simulink model "parcial_2_simulaciones"  (R2026a)
settings: Solver=VariableStepAuto
undefined symbols (not defined in the file): A, B, C, D
settings Model: Creator=santi  LastModifiedBy=elkin

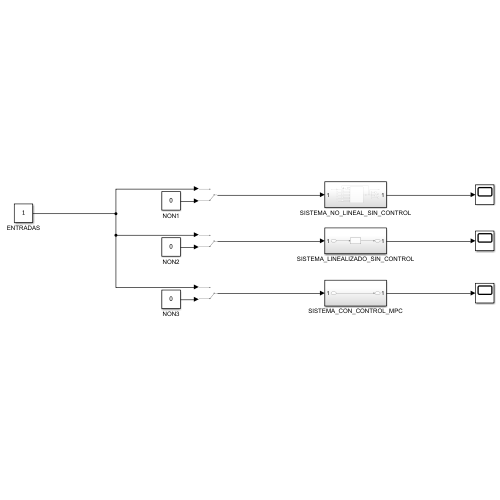
[thumbnail: Simulink's stored preview of the top-level diagram]
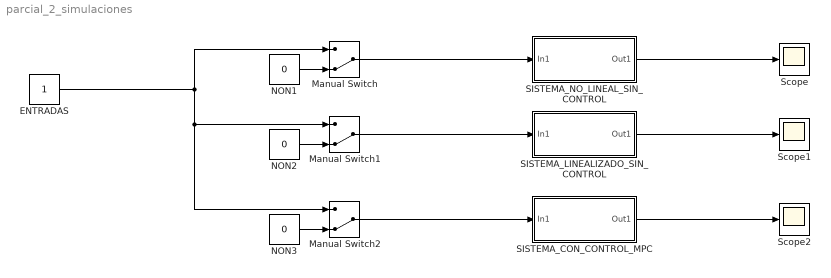
== system parcial_2_simulaciones ==
  ENTRADAS : Constant
  Manual Switch : ManualSwitch  CurrentSetting=0
  Manual Switch1 : ManualSwitch  CurrentSetting=0
  Manual Switch2 : ManualSwitch  CurrentSetting=0
  NON1 : Constant  Value=0
  NON2 : Constant  Value=0
  NON3 : Constant  Value=0
  SISTEMA_CON_CONTROL_MPC : Subsystem
  SISTEMA_LINEALIZADO_SIN_CONTROL : Subsystem
  SISTEMA_NO_LINEAL_SIN_CONTROL : Subsystem
  Scope : Scope
  Scope1 : Scope
      settings: ActiveDisplayYMinimum=-1.6528238285250998E+23  ActiveDisplayYMaximum=1.48754144567259E+24
  Scope2 : Scope
      settings: DataLoggingVariableName=ScopeData2
  wires:
  ENTRADAS/1 -> Manual Switch2/1, Manual Switch1/1, Manual Switch/1
  Manual Switch/1 -> SISTEMA_NO_LINEAL_SIN_CONTROL/1(In1)
  NON2/1 -> Manual Switch1/2
  NON1/1 -> Manual Switch/2
  NON3/1 -> Manual Switch2/2
  Manual Switch1/1 -> SISTEMA_LINEALIZADO_SIN_CONTROL/1(In1)
  Manual Switch2/1 -> SISTEMA_CON_CONTROL_MPC/1(In1)
  SISTEMA_NO_LINEAL_SIN_CONTROL/1(Out1) -> Scope/1
  SISTEMA_LINEALIZADO_SIN_CONTROL/1(Out1) -> Scope1/1
  SISTEMA_CON_CONTROL_MPC/1(Out1) -> Scope2/1

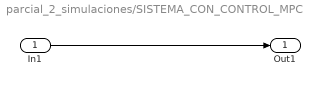
== system parcial_2_simulaciones/SISTEMA_CON_CONTROL_MPC ==
  In1 : Inport
  Out1 : Outport
  wires:
  In1/1 -> Out1/1

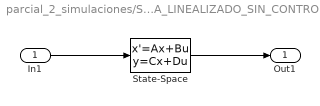
== system parcial_2_simulaciones/SISTEMA_LINEALIZADO_SIN_CONTROL ==
  In1 : Inport
  State-Space : StateSpace  A=A  B=B  C=C  D=D  InitialCondition=[0; 0; 0; 0]
  Out1 : Outport
  wires:
  In1/1 -> State-Space/1
  State-Space/1 -> Out1/1

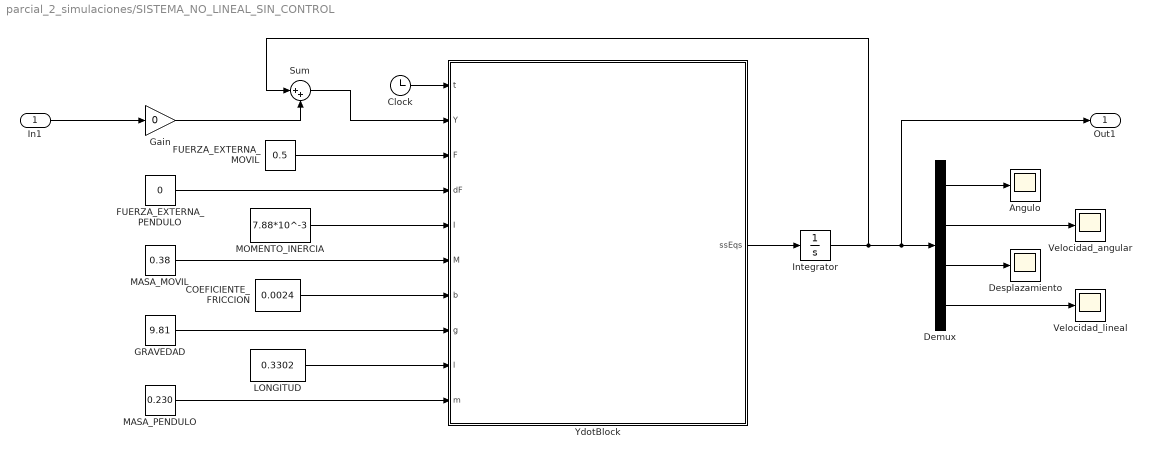
== system parcial_2_simulaciones/SISTEMA_NO_LINEAL_SIN_CONTROL ==
  In1 : Inport
  Angulo : Scope
      settings: ActiveDisplayYMinimum=-0.76325859502205173  ActiveDisplayYMaximum=6.8693273551984673  DataLoggingVariableName=ScopeData4
  COEFICIENTE_FRICCION : Constant  Value=0.0024
  Clock : Clock
  Demux : Demux
  Desplazamiento : Scope
      settings: ActiveDisplayYMinimum=-5.0622764494535364  ActiveDisplayYMaximum=45.560488045081833  DataLoggingVariableName=ScopeData5
  FUERZA_EXTERNA_MOVIL : Constant  Value=0.5
  FUERZA_EXTERNA_PENDULO : Constant  Value=0
  GRAVEDAD : Constant  Value=9.81
  Gain : Gain  Gain=0
  Integrator : Integrator
  LONGITUD : Constant  Value=0.3302
  MASA_MOVIL : Constant  Value=0.38
  MASA_PENDULO : Constant  Value=0.230
  MOMENTO_INERCIA : Constant  Value=7.88*10^-3
  Sum : Sum  Inputs=|++
  Velocidad_angular : Scope
      settings: ActiveDisplayYMinimum=-14.075103599955737  ActiveDisplayYMaximum=14.078691022077345  DataLoggingVariableName=ScopeData6
  Velocidad_lineal : Scope
      settings: ActiveDisplayYMinimum=-1.8590489212415653  ActiveDisplayYMaximum=9.7192759537899871  DataLoggingVariableName=ScopeData3
  YdotBlock : MATLAB Function  TreatAsAtomicUnit=on
  Out1 : Outport
  wires:
  YdotBlock/1(ssEqs) -> Integrator/1
  Demux/3 -> Desplazamiento/1
  MASA_PENDULO/1 -> YdotBlock/10(m)
  FUERZA_EXTERNA_MOVIL/1 -> YdotBlock/3(F)
  MASA_MOVIL/1 -> YdotBlock/6(M)
  Integrator/1 -> Sum/1, Out1/1, Demux/1
  Demux/2 -> Velocidad_angular/1
  LONGITUD/1 -> YdotBlock/9(l)
  Demux/4 -> Velocidad_lineal/1
  COEFICIENTE_FRICCION/1 -> YdotBlock/7(b)
  Demux/1 -> Angulo/1
  GRAVEDAD/1 -> YdotBlock/8(g)
  FUERZA_EXTERNA_PENDULO/1 -> YdotBlock/4(dF)
  Clock/1 -> YdotBlock/1(t)
  MOMENTO_INERCIA/1 -> YdotBlock/5(I)
  In1/1 -> Gain/1
  Gain/1 -> Sum/2
  Sum/1 -> YdotBlock/2(Y)

== matlab function parcial_2_simulaciones/SISTEMA_NO_LINEAL_SIN_CONTROL/YdotBlock ==
  data: t input; ssEqs output; Y input size=[4 1]; F input; dF input; I input; M input; b input; g input; l input; m input
function ssEqs = YdotBlock(t,Y,F,dF,I,M,b,g,l,m)
%#codegen

%    This function was generated by the Symbolic Math Toolbox version 25.1.
%    01-Nov-2026 18:24:22

% t = complex(t);  % if required to enforce complex operations
% Y = complex(Y);  % if required to enforce complex operations
% F = complex(F);  % if required to enforce complex operations
% dF = complex(dF);  % if required to enforce complex operations
% I = complex(I);  % if required to enforce complex operations
% M = complex(M);  % if required to enforce complex operations
% b = complex(b);  % if required to enforce complex operations
% g = complex(g);  % if required to enforce complex operations
% l = complex(l);  % if required to enforce complex operations
% m = complex(m);  % if required to enforce complex operations
t2 = I.*m;
t3 = Y(1);
t4 = Y(2);
t5 = Y(4);
t6 = l.^2;
t7 = m.^2;
t8 = I.*M;
t9 = cos(t3);
t10 = sin(t3);
t11 = t4.^2;
t13 = M.*m.*t6;
t14 = t6.*t7;
t12 = t9.^2;
t15 = t12.*t14;
t16 = -t15;
t17 = t2+t8+t13+t14+t16;
t18 = 1.0./t17;
ssEqs = [t4;l.*t18.*(M.*dF.*t9+F.*m.*t9+g.*t7.*t10-b.*m.*t5.*t9+M.*g.*m.*t10-l.*t7.*t9.*t10.*t11);t5;-t18.*(I.*dF-F.*I+I.*b.*t5-F.*m.*t6+dF.*m.*t6+b.*m.*t5.*t6-dF.*m.*t6.*t12-g.*t9.*t10.*t14+l.*t2.*t10.*t11+l.^3.*t7.*t10.*t11)];
end
